simulink model "UAM_Hexa_PD_Diff_SIL"  (R2026a)
settings: Solver=ode4  StopTime=tf  FixedStep=0.01
values from neighbouring files (symbols this model uses):
  ArmConstants = struct('l1_dim', l1_dim,                        'l2_dim', l2_dim,                        'Hexa_to_joint_L', L,                        'Mass1', ml1,                        'Mass2', ml2,                        'Inertia1', Hl1,                        'Inertia2', Hl2,                        'MC1', c1,                        'MC2', c2,                        'Servos', Servos)    [init_model.m]    (also in init_var.m)
settings Model: SILPILSystemUnderTest=refmodels  Creator=Carlos Fabian  LastModifiedBy=Carlos Fabian
settings OptimizationCC: UseDivisionForNetSlopeComputation=on
settings RTWCC: SystemTargetFile=ert.tlc  Description=Embedded Coder
settings ERTTargetCC: GenerateSampleERTMain=on
settings ExplorerConfigSet: InternalSimMechanicsExplorerSettings=|
  | <ExplorerConfiguration>
  | 
  |   <canonicalview>default</canonicalview>
  | 
  |   <TilePanel>
  |     <TileInfo>
  |       <Tiles Columns="1" Count="1" Height="513" Rows="1" Width="1199">
  |         <Row Weight="1"/>
  |         <Column Weight="1"/>
  |         <Tile Height="1" Width="1" X="0" Y="0"/>
  |       </Tiles>
  |     </TileInfo>
  |     <SceneInfo>
  |       <SceneViewer>
  |         <IsThisViewStd>
  |           <IsStandardView>off</IsStandardView>
  |           <StandardViewName>Front</StandardViewName>
  |         </IsThisViewStd>
  |         <BGColor>
  |           <R>1</R>
  |           <G>1</G>
  |           <B>1</B>
  |           <A>1</A>
  |         </BGColor>
  |         <Camera>
  |           <DoPerspective>off</DoPerspective>
  |           <Position>
  |             <X>16.563809413425133</X>
  |             <Y>-16.563809413425133</Y>
  |             <Z>17.346953838391503</Z>
  |           </Position>
  |           <Center>
  |             <X>0</X>
  |             <Y>0</Y>
  |             <Z>0.78314442496637693</Z>
  |           </Center>
  |           <Up>
  |             <X>-0.40824829046386285</X>
  |             <Y>0.40824829046386285</Y>
  |             <Z>0.81649658092772603</Z>
  |           </Up>
  |           <XLim>3.39184009237395</XLim>
  |           <YLim>3.39184009237395</YLim>
  |           <ViewLimDist>0.01</ViewLimDist>
  |         </Camera>
  |       </SceneViewer>
  |     </SceneInfo>
  |   </TilePanel>
  | 
  |   <MechEditorPanel>
  |     <GfxPanelCameraMap/>
  |     <Cameras/>
  |     <VideoCreator>
  |       <IncludeTiles>All</IncludeTiles>
  |       <IncludeTime>on</IncludeTime>
  |       <IncludeWorldFrame>off</IncludeWorldFrame>
  |       <PlaybackSpeedRatio>8</PlaybackSpeedRatio>
  |       <FrameRate>24</FrameRate>
  |       <FrameSize>auto</FrameSize>
  |       <VideoFormat>MotionJPEGAVI</VideoFormat>
  |     </VideoCreator>
  |   </MechEditorPanel>
  | 
  |   <PlaybackSettings>
  |     <PlaybackSpeedFactor>4</PlaybackSpeedFactor>
  |   </PlaybackSettings>
  | 
  | </ExplorerConfiguration>

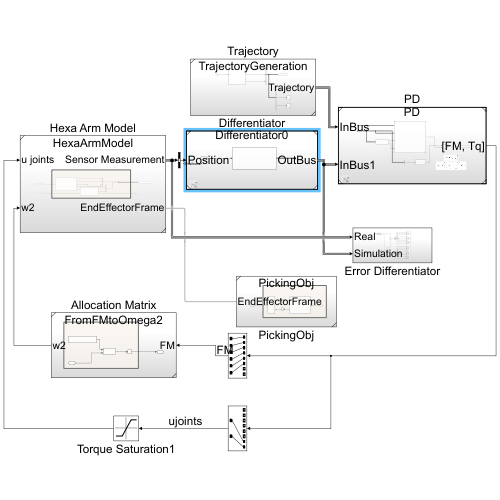
[thumbnail: Simulink's stored preview of the top-level diagram]
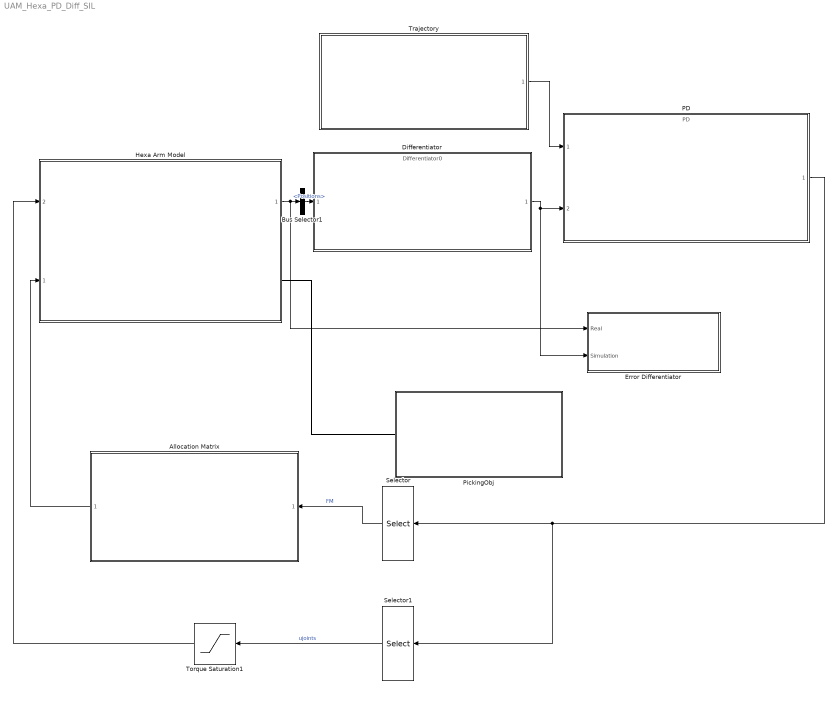
== system UAM_Hexa_PD_Diff_SIL ==
  Allocation Matrix : Subsystem  ReferencedSubsystem=FromFMtoOmega2
  Bus Selector1 : BusSelector  OutputSignals=Positions
  Differentiator : ModelReference  ModelNameDialog=Differentiator0  SimulationMode=Normal  ModelReferenceVersion=1.68
  Error Differentiator : Subsystem
  Hexa Arm Model : Subsystem  ReferencedSubsystem=HexaArmModel
      settings: PortSchema="{\"entries\":[{\"content\":{\"sides\":[{\"content\":{\"connectorIds\":[\"In2\",\"In1\"]},\"type\":\"ConnectorPlacement.EquallySpacedRectSide\",\"uuid\":\"8c321911-c61a-4c60-b031-eeaf4c8b5083\"},{\"content\":{\"connectorIds\":[\"Out1\",\"RConn1\"],\"side\":\"RIGHT\"},\"type\":\"ConnectorPlacement.EquallySpacedRectSide\",\"uuid\":\"3ad1588f-e2f8-4666-8b86-318f5207193d\"},{\"content\":{\"side\":\"TOP\"},\"type\":\"ConnectorPlacement.EquallySpacedRectSide\",\"uuid\":\"710cc49c-59c4-4f69-a558-4588d1d119c0\"}]},\"type\":\"ConnectorPlacement.EquallySpacedConnector\",\"uuid\":\"3e8cca1f-f7f1-4f31-9eba-ef93ff8e81e8\"}],\"packageUris\":[\"http://schema.mathworks.com/mf0/Connector/R2020b\"],\"version\":\"1.0\"}"
  PD : ModelReference  ModelNameDialog=PD  SimulationMode=Normal  CodeInterface=Top model  ModelReferenceVersion=1.69
  PickingObj : Subsystem  ReferencedSubsystem=PickingObj
  Selector : Selector  InputPortWidth=8  IndexOptions=Index vector (dialog)  Indices=1:6  OutputSizes=1
  Selector1 : Selector  InputPortWidth=8  IndexOptions=Index vector (dialog)  Indices=7:8  OutputSizes=1
  Torque Saturation1 : Saturate  UpperLimit=ArmConstants.Servos.T1max  LowerLimit=-ArmConstants.Servos.T1max
  Trajectory : Subsystem  ReferencedSubsystem=TrajectoryGeneration
  wires:
  Selector/1 -> Allocation Matrix/1  "FM"
  PD/1 -> Selector/1, Selector1/1
  Torque Saturation1/1 -> Hexa Arm Model/2
  Selector1/1 -> Torque Saturation1/1  "ujoints"
  Trajectory/1 -> PD/1
  Allocation Matrix/1 -> Hexa Arm Model/1
  Hexa Arm Model/1 -> Error Differentiator/1(Real), Bus Selector1/1
  Differentiator/1 -> Error Differentiator/2(Simulation), PD/2
  Bus Selector1/1 -> Differentiator/1  "<Positions>"
  connections:
  Hexa Arm Model/RConn1 -- PickingObj/LConn1

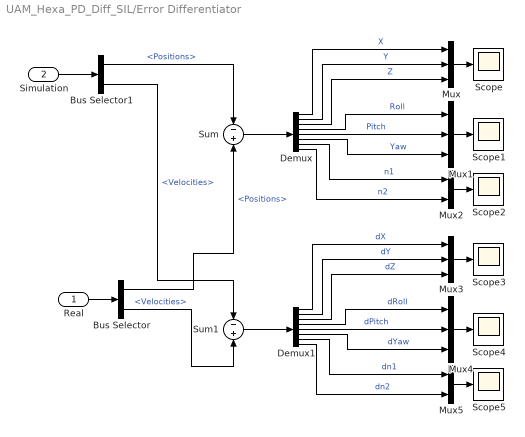
== system UAM_Hexa_PD_Diff_SIL/Error Differentiator ==
  Real : Inport
  Simulation : Inport  Port=2
  Bus Selector : BusSelector  OutputSignals=Positions,Velocities
  Bus Selector1 : BusSelector  OutputSignals=Positions,Velocities
  Demux : Demux  Outputs=8
  Demux1 : Demux  Outputs=8
  Mux{,1,3..4} (4 alike) : Mux  Inputs=3
  Mux2 : Mux  Inputs=2
  Mux5 : Mux  Inputs=2
  Scope{,1..5} (6 alike) : Scope
      Scope settings: ActiveDisplayYMinimum=-0.11516314203526654  ActiveDisplayYMaximum=0.12253392651728615
      Scope1 settings: ActiveDisplayYMinimum=-0.039456080037096539  ActiveDisplayYMaximum=0.028206770020752458  DataLoggingVariableName=ScopeData4
      Scope2 settings: ActiveDisplayYMinimum=-0.097057334019579361  ActiveDisplayYMaximum=0.091379254090405648  DataLoggingVariableName=ScopeData5
      Scope3 settings: ActiveDisplayYMinimum=-0.12118491948489385  ActiveDisplayYMaximum=0.25198076657940688  DataLoggingVariableName=ScopeData6
      Scope4 settings: ActiveDisplayYMinimum=-0.049702476607807689  ActiveDisplayYMaximum=0.057495988286683834  DataLoggingVariableName=ScopeData7
      Scope5 settings: ActiveDisplayYMinimum=-11.414042765802602  ActiveDisplayYMaximum=7.1811721637788093  DataLoggingVariableName=ScopeData8
  Sum : Sum  Inputs=-+
  Sum1 : Sum  Inputs=-+
  wires:
  Mux2/1 -> Scope2/1
  Sum/1 -> Demux/1
  Mux1/1 -> Scope1/1
  Bus Selector1/1 -> Sum/1  "<Positions>"
  Demux/8 -> Mux2/2  "n2"
  Bus Selector/2 -> Sum1/2  "<Velocities>"
  Demux/7 -> Mux2/1  "n1"
  Mux/1 -> Scope/1
  Demux/1 -> Mux/1  "X"
  Demux/4 -> Mux1/1  "Roll"
  Demux/6 -> Mux1/3  "Yaw"
  Demux/5 -> Mux1/2  "Pitch"
  Demux/3 -> Mux/3  "Z"
  Bus Selector/1 -> Sum/2  "<Positions>"
  Demux/2 -> Mux/2  "Y"
  Bus Selector1/2 -> Sum1/1  "<Velocities>"
  Simulation/1 -> Bus Selector1/1
  Real/1 -> Bus Selector/1
  Demux1/8 -> Mux5/2  "dn2"
  Mux4/1 -> Scope4/1
  Sum1/1 -> Demux1/1
  Mux5/1 -> Scope5/1
  Demux1/4 -> Mux4/1  "dRoll"
  Demux1/6 -> Mux4/3  "dYaw"
  Demux1/2 -> Mux3/2  "dY"
  Demux1/1 -> Mux3/1  "dX"
  Mux3/1 -> Scope3/1
  Demux1/5 -> Mux4/2  "dPitch"
  Demux1/7 -> Mux5/1  "dn1"
  Demux1/3 -> Mux3/3  "dZ"
